simulink model "tg9"  (R2022a)
settings: Solver=ode15s  StartTime=0.0  StopTime=10  MaxStep=0.01  RelTol=1e-3
InitFcn:
  | mecha_param2
  | control_param0
values from neighbouring files (symbols this model uses):
  b0 = 0    [sim_IMMC.m]
  b1 = 1    [sim_IMMC.m]
  back0 = 0    [sim_IMMC.m]
  back1 = 0    [sim_IMMC.m]
  boff = 0    [sim_IMMC.m]
  bon = 0    [sim_IMMC.m]
  c = 0.05    [mecha_param2.m]
  c_jointstop = 0.3 / (pi/180)    (= 17.1887338539)    [mecha_param2.m]
  calctalus = sqrt((L_foot - (DJ1x_foot))^2 + (H_foot-r_cs)^2)    [mecha_param2.m]
  calctoes = sqrt((H_foot-r_cs)^2 + (DJ1x_foot)^2)    [mecha_param2.m]
  corrD = 0.001    [control_param0.m]
  DG_HAT = 0.35    [mecha_param2.m]
  DG_thigh = 0.28    [mecha_param2.m]
  DJ1x_foot = 0.16-r_cs    (= 0.135)    [mecha_param2.m]
  eref = 0.04    [mecha_param2.m]
  FmaxBFSH = 350    [mecha_param2.m]
  FmaxGAS = 1500    [mecha_param2.m]
  FmaxGLU = 1500    [mecha_param2.m]
  FmaxHAM = 3000    [mecha_param2.m]
  FmaxHFL = 2000    [mecha_param2.m]
  FmaxRF = 1200    [mecha_param2.m]
  FmaxSOL = 4000    [mecha_param2.m]
  FmaxTA = 800    [mecha_param2.m]
  FmaxVAS = 6000    [mecha_param2.m]
  g = 9.81    [mecha_param2.m]
  g0 = 0    [sim_IMMC.m]
  g1 = 0    [sim_IMMC.m]
  H_foot = 0.08    [mecha_param2.m]
  In_HAT = 3    [mecha_param2.m]
  In_shank = 0.05    [mecha_param2.m]
  In_thigh = 0.15    [mecha_param2.m]
  K = 5    [mecha_param2.m]
  knee_thigh = [0 0 -(L_thigh/2)]    [mecha_param2.m]
  Kpress = m_HAT * g / DeltaThRef    (= 104967)    [mecha_param2.m]
  L_foot = 0.2    [mecha_param2.m]
  L_HAT = 0.8    [mecha_param2.m]
  L_shank = 0.46    [mecha_param2.m]
  L_thigh = 0.46    [mecha_param2.m]
  LoHAM = table2array(mt('LoHAM', 1))    [control_param0.m]
  LoHFL = table2array(mt('LoHFL', 1))    [control_param0.m]
  longD = longD - corrD    (= 0.019)    [control_param0.m]
  loptBFSH = 0.12    [mecha_param2.m]
  loptGAS = 0.05    [mecha_param2.m]
  loptGLU = 0.11    [mecha_param2.m]
  loptHAM = 0.10    (= 0.1)    [mecha_param2.m]
  loptHFL = 0.11    [mecha_param2.m]
  loptRF = 0.08    [mecha_param2.m]
  loptSOL = 0.04    [mecha_param2.m]
  loptTA = 0.06    [mecha_param2.m]
  loptVAS = 0.08    [mecha_param2.m]
  LoTA = table2array(mt('LoTA', 1))    [control_param0.m]
  lslackBFSH = 0.10    (= 0.1)    [mecha_param2.m]
  lslackGAS = 0.40    (= 0.4)    [mecha_param2.m]
  lslackGLU = 0.13    [mecha_param2.m]
  lslackHAM = 0.31    [mecha_param2.m]
  lslackHFL = 0.10    (= 0.1)    [mecha_param2.m]
  lslackRF = 0.35    [mecha_param2.m]
  lslackSOL = 0.26    [mecha_param2.m]
  lslackTA = 0.24    [mecha_param2.m]
  lslackVAS = 0.23    [mecha_param2.m]
  m_HAT = 53.5    [mecha_param2.m]
  m_shank = 3.5    [mecha_param2.m]
  m_thigh = 8.5    [mecha_param2.m]
  midD = midD - corrD    (= 0.009)    [control_param0.m]
  N = 1.5    [mecha_param2.m]
  nonoff = 0    [control_param0.m]
  phi_a_low = (70) * (pi / 180)    (= 1.2217304764)    [mecha_param2.m]
  phi_a_up = (130) * (pi / 180)    (= 2.26892802759)    [mecha_param2.m]
  phi_dl = 180    [mecha_param2.m]
  phi_h = 230 * (pi / 180)    (= 4.01425727959)    [mecha_param2.m]
  phi_k = 175 * (pi / 180)    (= 3.05432619099)    [mecha_param2.m]
  phictoes = asind((DJ1y_foot-r_cs)/calctoes)    [mecha_param2.m]
  phimaxGASa = 100*pi/180    (= 1.74532925199)    [mecha_param2.m]
  phimaxGASk = 140*pi/180    (= 2.44346095279)    [mecha_param2.m]
  phimaxRFk = 165*pi/180    (= 2.87979326579)    [mecha_param2.m]
  phimaxSOL = 100*pi/180    (= 1.74532925199)    [mecha_param2.m]
  phimaxTA = 80*pi/180    (= 1.3962634016)    [mecha_param2.m]
  phimaxVAS = 165*pi/180    (= 2.87979326579)    [mecha_param2.m]
  phirefBFSH = 160*pi/180    (= 2.79252680319)    [mecha_param2.m]
  phirefGASa = 80*pi/180    (= 1.3962634016)    [mecha_param2.m]
  phirefGASk = 165*pi/180    (= 2.87979326579)    [mecha_param2.m]
  phirefGLU = 120*pi/180    (= 2.09439510239)    [mecha_param2.m]
  phirefHAMh = 150*pi/180    (= 2.61799387799)    [mecha_param2.m]
  phirefHAMk = 180*pi/180    (= 3.14159265359)    [mecha_param2.m]
  phirefHFL = 160*pi/180    (= 2.79252680319)    [mecha_param2.m]
  phirefRFh = 170*pi/180    (= 2.96705972839)    [mecha_param2.m]
  phirefRFk = 125*pi/180    (= 2.18166156499)    [mecha_param2.m]
  phirefSOL = 90*pi/180    (= 1.57079632679)    [mecha_param2.m]
  phirefTA = 110*pi/180    (= 1.91986217719)    [mecha_param2.m]
  phirefVAS = 120*pi/180    (= 2.09439510239)    [mecha_param2.m]
  phiScaleGASa = acos(rGASamin/rGASamax)/(phiminGASa-phimaxGASa)    [mecha_param2.m]
  phiScaleGASk = acos(rGASkmin/rGASkmax)/(phiminGASk-phimaxGASk)    [mecha_param2.m]
  phiScaleRFk = acos(rRFkmin/rRFkmax)/(phiminRFk-phimaxRFk)    [mecha_param2.m]
  phiScaleSOL = acos(rSOLmin/rSOLmax)/(phiminSOL-phimaxSOL)    [mecha_param2.m]
  phiScaleTA = acos(rTAmin/rTAmax)/(phiminTA-phimaxTA)    [mecha_param2.m]
  phiScaleVAS = acos(rVASmin/rVASmax)/(phiminVAS-phimaxVAS)    [mecha_param2.m]
  r1 = 0    [sim_IMMC.m]
  r_cs = 0.025    [mecha_param2.m]
  rBFSH = 0.04    [mecha_param2.m]
  rGASamax = 0.06    [mecha_param2.m]
  rGASkmax = 0.05    [mecha_param2.m]
  rGLU = 0.08    [mecha_param2.m]
  rHAMh = 0.08    [mecha_param2.m]
  rHAMk = 0.05    [mecha_param2.m]
  rHFL = 0.08    [mecha_param2.m]
  rhoBFSH = 0.7    [mecha_param2.m]
  rhoGASa = 0.7    [mecha_param2.m]
  rhoGASk = 0.7    [mecha_param2.m]
  rhoGLU = 0.5    [mecha_param2.m]
  rhoHAMh = 0.5    [mecha_param2.m]
  rhoHAMk = 0.5    [mecha_param2.m]
  rhoHFL = 0.5    [mecha_param2.m]
  rhoRFh = 0.3    [mecha_param2.m]
  rhoRFk = 0.5    [mecha_param2.m]
  rhoSOL = 0.5    [mecha_param2.m]
  rhoTA = 0.7    [mecha_param2.m]
  rhoVAS = 0.6    [mecha_param2.m]
  rRFh = 0.08    [mecha_param2.m]
  rRFkmax = 0.06    [mecha_param2.m]
  rSOLmax = 0.06    [mecha_param2.m]
  ... (+25 more)
undefined symbols (not defined in the file or in its folder): beta11, beta12, beta13, beta14, beta15, beta16, beta21, beta22, beta23, beta24, beta25, beta26, beta31, beta32, beta33, beta34, beta35, beta36, beta41, beta42, beta43, beta44, beta45, beta46, beta51, beta52, beta53, beta54, beta55, beta56, betab1, betab2, betab3, betab4, betab5, betab6, betap11, betap12, betap13, betap14, betap15, betap16, betap21, betap22, betap23, betap24, betap25, betap26, betap31, betap32, betap33, betap34, betap35, betap36, betap41, betap42, betap43, betap44, betap45, betap46 ... (+102)
libraries: sm_lib x89, simulink x72, nesl_utility x58, simulink_extras x18
(part 6 of 12)

== system tg9/Muscle Actuation Layer/L Ankle Joint Limit ==
  note: Right Ankle Soft Limit
  phi [rad] : Inport
  dphi [rad/s] : Inport  Port=2
  Gain : Gain  Gain=c_jointstop
  Gain1 : Gain  Gain=1/w_max_jointstop
  Gain2 : Gain  Gain=-1
  Gain3 : Gain  Gain=c_jointstop
  Interval Test : simulink/Logic and Bit Operations/Interval Test  IntervalClosedRight=on  uplimit=phi_a_up + 40*pi/180  IntervalClosedLeft=on  lowlimit=phi_a_low - 40*pi/180  OutDataTypeStr=boolean
  Logical Operator : Logic  Operator=NOT  AllPortsSameDT=off  OutDataTypeStr=boolean
  Mux : Mux  Inputs=2
  Mux1 : Mux  Inputs=2
  Overextension torque : MATLAB Function  TreatAsAtomicUnit=on
  Overflexion torque : MATLAB Function  TreatAsAtomicUnit=on
  Scope : Scope
  Scope1 : Scope  NumInputPorts=2
  Stop Simulation : Stop
  Sum : Sum  Inputs=|+-
  Sum1 : Sum  Inputs=|+-
  Sum2 : Sum  Inputs=+|+
  overextension angle : Constant  Value=phi_a_up
  overflexion angle : Constant  Value=phi_a_low
  M_stop [Nm] : Outport
  wires:
  phi [rad]/1 -> Sum/1, Interval Test/1, Sum1/1
  overextension angle/1 -> Sum/2
  dphi [rad/s]/1 -> Gain1/1
  Sum/1 -> Gain/1
  Gain1/1 -> Mux1/2, Gain2/1
  Gain/1 -> Mux/1
  Gain2/1 -> Mux/2
  Mux/1 -> Overextension torque/1(u)
  Interval Test/1 -> Logical Operator/1
  Logical Operator/1 -> Scope/1, Stop Simulation/1
  Gain3/1 -> Mux1/1
  Sum1/1 -> Gain3/1
  overflexion angle/1 -> Sum1/2
  Overflexion torque/1(y) -> Sum2/2, Scope1/2
  Mux1/1 -> Overflexion torque/1(u)
  Overextension torque/1(y) -> Scope1/1, Sum2/1
  Sum2/1 -> M_stop [Nm]/1

== system tg9/Muscle Actuation Layer/L BFSH ==
  note: fv
  note: STIM to A
  note: v[vmax] becomes v when *vmax and vce when *lopt
  note: lce is the integration of vce over time using lopt as initial condition
  note: vce
  note: activation
  note: stimulation
  note: Fmax
  note: Fmtc = Fse
  note: outcome fse is a proportion of fmax, because of that, it must be multiplied by fmax in order to get Fse
  note: lceo = lmtu-lslack
  note: lse=lmtu-lce
  note: lse/lslack
  note: lce/lopt
  note: lce
  note: lce
  note: lce
  note: lmtu
  note: lmtu
  note: Left Biceps femoris short-head Musculo-Tendon Unit
  STIM : Inport
  lmtu [m] : Inport  Port=2
  BE force-length relation : Subsystem
  CE force-length relation : Subsystem
  CE inverse force-velocity relation : Subsystem
  Constant : Constant  Value=lslackBFSH
  ECC TransferFcn : simulink_extras/Additional Linear/Transfer Fcn (with initial outputs)  N=[1]  D="[tau  1]"  Y0=preA  U0=0
  Fv = (Fse+Fbe) / (A*Fce+Fpe) : Product  Inputs=*/
  Gain : Gain  Gain=vmaxBFSH*loptBFSH
  Gain1 : Gain  Gain=1/lslackBFSH
  Gain2 : Gain  Gain=1/loptBFSH
  Gain3 : Gain  Gain=FmaxBFSH
  Integrator : Integrator  InitialConditionSource=external  ZeroCross=off
  PE force-length relation : Subsystem
  Product : Product
  SE force-length relation : Subsystem
  Sum : Sum  Inputs=|+-
  Sum1 : Sum  Inputs=|-+
  Sum2 : Sum  Inputs=+|+
  Sum3 : Sum  Inputs=+|+
  excentric branch1 : Fcn  Commented=on  Expr=u(2) * (u(1)>1)*(u(1)<=u(3))
  Fmtc : Outport
  Lce : Outport  Port=2
  Vce : Outport  Port=3
  lse : Outport  Port=4
  A : Outport  Port=5
  fce [Fmax] : Outport  Port=6
  "fse [Fmax}" : Outport  Port=7
  wires:
  CE inverse force-velocity relation/1(v[vmax]) -> Gain/1
  PE force-length relation/1(fpe [Fmax]) -> Sum3/1
  BE force-length relation/1(fbe [Fmax]) -> Sum2/2
  Fv = (Fse+Fbe) / (A*Fce+Fpe)/1 -> CE inverse force-velocity relation/1(Fv[Fmax])
  Sum3/1 -> Fv = (Fse+Fbe) / (A*Fce+Fpe)/2
  Sum2/1 -> Fv = (Fse+Fbe) / (A*Fce+Fpe)/1
  Gain3/1 -> Fmtc/1
  ECC TransferFcn/1 -> Product/2, A/1
  STIM/1 -> ECC TransferFcn/1
  Product/1 -> Sum3/2
  CE force-length relation/1(fce [Fmax]) -> Product/1, fce [Fmax]/1
  SE force-length relation/1(fse [Fmax]) -> Sum2/1, Gain3/1, "fse [Fmax}"/1
  Gain1/1 -> SE force-length relation/1(lse [lslack])
  Gain2/1 -> CE force-length relation/1(lce [lopt]), BE force-length relation/1(lce [lopt]), PE force-length relation/1(lce [lopt])
  Sum/1 -> Gain1/1, lse/1
  Gain/1 -> Integrator/1, Vce/1
  Sum1/1 -> Integrator/2
  Constant/1 -> Sum1/1
  Integrator/1 -> Lce/1, Gain2/1, Sum/2
  lmtu [m]/1 -> Sum/1, Sum1/2

== system tg9/Muscle Actuation Layer/L BFSH Link1 ==
  note: BFSH Attachment
  phi23 [rad] : Inport
  Constant : Constant  Value=lslackBFSH+loptBFSH
  Constant1 : Constant  Value=rBFSH
  Constant2 : Constant  Value=phirefBFSH
  Gain4 : Gain  Gain=rhoBFSH
  Product : Product  RndMeth=Zero
  Sum2 : Sum  Inputs=|+-
  Sum5 : Sum  Inputs=|++
  lmtu [m] : Outport
  lever [m] : Outport  Port=2
  wires:
  Constant/1 -> Sum5/1
  Sum5/1 -> lmtu [m]/1
  Gain4/1 -> Sum5/2
  Product/1 -> Gain4/1
  phi23 [rad]/1 -> Sum2/1
  Constant2/1 -> Sum2/2
  Sum2/1 -> Product/1
  Constant1/1 -> Product/2, lever [m]/1

== system tg9/Muscle Actuation Layer/L BFSH Link2 ==
  note: BFSH Attachment
  phi23 [rad] : Inport
  Constant : Constant  Value=lslackBFSH+loptBFSH
  Constant1 : Constant  Value=rBFSH
  Constant2 : Constant  Value=phirefBFSH
  Gain4 : Gain  Gain=rhoBFSH
  Product : Product  RndMeth=Zero
  Sum2 : Sum  Inputs=|+-
  Sum5 : Sum  Inputs=|++
  lmtu [m] : Outport
  lever [m] : Outport  Port=2
  wires:
  Constant/1 -> Sum5/1
  Sum5/1 -> lmtu [m]/1
  Gain4/1 -> Sum5/2
  Product/1 -> Gain4/1
  phi23 [rad]/1 -> Sum2/1
  Constant2/1 -> Sum2/2
  Sum2/1 -> Product/1
  Constant1/1 -> Product/2, lever [m]/1

== system tg9/Muscle Actuation Layer/L GAS ==
  note: Left Gastrocnemius Musculo-Tendon Unit
  note: lmtu
  note: lmtu
  note: lce
  note: lce
  note: lce
  note: lce/lopt
  note: lse/lslack
  note: lse=lmtu-lce
  note: lceo = lmtu-lslack
  note: outcome fse is a proportion of fmax, because of that, it must be multiplied by fmax in order to get Fse
  note: Fmtc = Fse
  note: Fmax
  note: stimulation
  note: activation
  note: vce
  note: lce is the integration of vce over time using lopt as initial condition
  note: v[vmax] becomes v when *vmax and vce when *lopt
  note: STIM to A
  note: fv
  STIM : Inport
  lmtu [m] : Inport  Port=2
  BE force-length relation : Subsystem
  CE force-length relation : Subsystem
  CE inverse force-velocity relation : Subsystem
  Constant : Constant  Value=lslackGAS
  ECC TransferFcn : simulink_extras/Additional Linear/Transfer Fcn (with initial outputs)  N=[1]  D="[tau  1]"  Y0=preA  U0=0
  Fv = (Fse+Fbe) / (A*Fce+Fpe) : Product  Inputs=*/
  Gain : Gain  Gain=vmaxGAS*loptGAS
  Gain1 : Gain  Gain=1/lslackGAS
  Gain2 : Gain  Gain=1/loptGAS
  Gain3 : Gain  Gain=FmaxGAS
  Integrator : Integrator  InitialConditionSource=external  ZeroCross=off
  PE force-length relation : Subsystem
  Product : Product
  SE force-length relation : Subsystem
  Sum : Sum  Inputs=|+-
  Sum1 : Sum  Inputs=|-+
  Sum2 : Sum  Inputs=+|+
  Sum3 : Sum  Inputs=+|+
  excentric branch1 : Fcn  Commented=on  Expr=u(2) * (u(1)>1)*(u(1)<=u(3))
  Fmtc : Outport
  Lce : Outport  Port=2
  Vce : Outport  Port=3
  lse : Outport  Port=4
  A : Outport  Port=5
  fce [Fmax] : Outport  Port=6
  "fse [Fmax}" : Outport  Port=7
  wires:
  lmtu [m]/1 -> Sum1/2, Sum/1
  Integrator/1 -> Sum/2, Gain2/1, Lce/1
  Constant/1 -> Sum1/1
  Sum1/1 -> Integrator/2
  Gain/1 -> Vce/1, Integrator/1
  Sum/1 -> lse/1, Gain1/1
  Gain2/1 -> PE force-length relation/1(lce [lopt]), BE force-length relation/1(lce [lopt]), CE force-length relation/1(lce [lopt])
  Gain1/1 -> SE force-length relation/1(lse [lslack])
  SE force-length relation/1(fse [Fmax]) -> "fse [Fmax}"/1, Gain3/1, Sum2/1
  CE force-length relation/1(fce [Fmax]) -> Product/1, fce [Fmax]/1
  Product/1 -> Sum3/2
  STIM/1 -> ECC TransferFcn/1
  ECC TransferFcn/1 -> A/1, Product/2
  Gain3/1 -> Fmtc/1
  Sum2/1 -> Fv = (Fse+Fbe) / (A*Fce+Fpe)/1
  Sum3/1 -> Fv = (Fse+Fbe) / (A*Fce+Fpe)/2
  Fv = (Fse+Fbe) / (A*Fce+Fpe)/1 -> CE inverse force-velocity relation/1(Fv[Fmax])
  BE force-length relation/1(fbe [Fmax]) -> Sum2/2
  PE force-length relation/1(fpe [Fmax]) -> Sum3/1
  CE inverse force-velocity relation/1(v[vmax]) -> Gain/1

== system tg9/Muscle Actuation Layer/L GAS Link1 ==
  note: GAS Attachment
  phi23 [rad] : Inport
  phi12 [rad] : Inport  Port=2
  Constant1 : Constant  Value=phimaxGASk
  Constant2 : Constant  Value=phirefGASk
  Constant3 : Constant  Value=phimaxGASa
  Constant4 : Constant  Value=lslackGAS+loptGAS
  Constant5 : Constant  Value=phirefGASa
  Demux : Demux  Outputs=2
  Demux1 : Demux  Outputs=2
  Gain1 : Gain  Gain=rGASkmax
  Gain2 : Gain  Gain=rGASamax
  Gain3 : Gain  Gain=phiScaleGASa
  Gain5 : Gain  Gain=phiScaleGASk
  Gain6 : Gain  Gain=phiScaleGASk
  Gain7 : Gain  Gain=rhoGASk/phiScaleGASk
  Gain8 : Gain  Gain=phiScaleGASa
  Gain9 : Gain  Gain=rhoGASa/phiScaleGASa
  Mux : Mux  Inputs=2
  Mux1 : Mux  Inputs=2
  Sum1 : Sum  Inputs=-+
  Sum2 : Sum  Inputs=|+-
  Sum3 : Sum  Inputs=-+|
  Sum4 : Sum  Inputs=-+
  Sum5 : Sum  Inputs=++-
  Sum6 : Sum  Inputs=|+-
  Sum7 : Sum  Inputs=-+|
  length change term : Trigonometry
  length change term1 : Trigonometry
  offset correction term : Trigonometry
  offset correction term1 : Trigonometry
  variable lever term : Trigonometry  Operator=cos
  variable lever term1 : Trigonometry  Operator=cos
  lmtu [m] : Outport
  lever23 [m] : Outport  Port=2
  lever12 [m] : Outport  Port=3
  wires:
  Sum5/1 -> lmtu [m]/1
  Demux1/2 -> lever12 [m]/1
  Constant4/1 -> Sum5/2
  Demux1/1 -> Gain9/1
  Gain9/1 -> Sum5/3
  Demux/2 -> lever23 [m]/1
  Demux/1 -> Gain7/1
  Gain7/1 -> Sum5/1
  phi23 [rad]/1 -> Sum3/2
  Sum3/1 -> Gain5/1
  Constant1/1 -> Sum3/1, Sum2/2
  Sum2/1 -> Gain6/1
  Constant2/1 -> Sum2/1
  length change term/1 -> Sum1/2
  offset correction term/1 -> Sum1/1
  Sum1/1 -> Mux/1
  variable lever term/1 -> Mux/2
  Mux/1 -> Gain1/1
  Gain1/1 -> Demux/1
  Gain5/1 -> variable lever term/1, length change term/1
  Gain6/1 -> offset correction term/1
  phi12 [rad]/1 -> Sum7/2
  Sum7/1 -> Gain3/1
  Constant3/1 -> Sum7/1, Sum6/2
  Sum6/1 -> Gain8/1
  Constant5/1 -> Sum6/1
  length change term1/1 -> Sum4/2
  offset correction term1/1 -> Sum4/1
  Sum4/1 -> Mux1/1
  variable lever term1/1 -> Mux1/2
  Mux1/1 -> Gain2/1
  Gain2/1 -> Demux1/1
  Gain3/1 -> variable lever term1/1, length change term1/1
  Gain8/1 -> offset correction term1/1

== system tg9/Muscle Actuation Layer/L GAS Link2 ==
  note: GAS Attachment
  phi23 [rad] : Inport
  phi12 [rad] : Inport  Port=2
  Constant1 : Constant  Value=phimaxGASk
  Constant2 : Constant  Value=phirefGASk
  Constant3 : Constant  Value=phimaxGASa
  Constant4 : Constant  Value=lslackGAS+loptGAS
  Constant5 : Constant  Value=phirefGASa
  Demux : Demux  Outputs=2
  Demux1 : Demux  Outputs=2
  Gain1 : Gain  Gain=rGASkmax
  Gain2 : Gain  Gain=rGASamax
  Gain3 : Gain  Gain=phiScaleGASa
  Gain5 : Gain  Gain=phiScaleGASk
  Gain6 : Gain  Gain=phiScaleGASk
  Gain7 : Gain  Gain=rhoGASk/phiScaleGASk
  Gain8 : Gain  Gain=phiScaleGASa
  Gain9 : Gain  Gain=rhoGASa/phiScaleGASa
  Mux : Mux  Inputs=2
  Mux1 : Mux  Inputs=2
  Sum1 : Sum  Inputs=-+
  Sum2 : Sum  Inputs=|+-
  Sum3 : Sum  Inputs=-+|
  Sum4 : Sum  Inputs=-+
  Sum5 : Sum  Inputs=++-
  Sum6 : Sum  Inputs=|+-
  Sum7 : Sum  Inputs=-+|
  length change term : Trigonometry
  length change term1 : Trigonometry
  offset correction term : Trigonometry
  offset correction term1 : Trigonometry
  variable lever term : Trigonometry  Operator=cos
  variable lever term1 : Trigonometry  Operator=cos
  lmtu [m] : Outport
  lever23 [m] : Outport  Port=2
  lever12 [m] : Outport  Port=3
  wires:
  Sum5/1 -> lmtu [m]/1
  Demux1/2 -> lever12 [m]/1
  Constant4/1 -> Sum5/2
  Demux1/1 -> Gain9/1
  Gain9/1 -> Sum5/3
  Demux/2 -> lever23 [m]/1
  Demux/1 -> Gain7/1
  Gain7/1 -> Sum5/1
  phi23 [rad]/1 -> Sum3/2
  Sum3/1 -> Gain5/1
  Constant1/1 -> Sum3/1, Sum2/2
  Sum2/1 -> Gain6/1
  Constant2/1 -> Sum2/1
  length change term/1 -> Sum1/2
  offset correction term/1 -> Sum1/1
  Sum1/1 -> Mux/1
  variable lever term/1 -> Mux/2
  Mux/1 -> Gain1/1
  Gain1/1 -> Demux/1
  Gain5/1 -> variable lever term/1, length change term/1
  Gain6/1 -> offset correction term/1
  phi12 [rad]/1 -> Sum7/2
  Sum7/1 -> Gain3/1
  Constant3/1 -> Sum7/1, Sum6/2
  Sum6/1 -> Gain8/1
  Constant5/1 -> Sum6/1
  length change term1/1 -> Sum4/2
  offset correction term1/1 -> Sum4/1
  Sum4/1 -> Mux1/1
  variable lever term1/1 -> Mux1/2
  Mux1/1 -> Gain2/1
  Gain2/1 -> Demux1/1
  Gain3/1 -> variable lever term1/1, length change term1/1
  Gain8/1 -> offset correction term1/1

== system tg9/Muscle Actuation Layer/L GLU ==
  note: Left Gluteus Musculo-Tendon Unit
  note: lmtu
  note: lmtu
  note: lce
  note: lce
  note: lce
  note: lce/lopt
  note: lse/lslack
  note: lse=lmtu-lce
  note: lceo = lmtu-lslack
  note: outcome fse is a proportion of fmax, because of that, it must be multiplied by fmax in order to get Fse
  note: Fmtc = Fse
  note: Fmax
  note: stimulation
  note: activation
  note: vce
  note: lce is the integration of vce over time using lopt as initial condition
  note: v[vmax] becomes v when *vmax and vce when *lopt
  note: STIM to A
  note: fv
  STIM : Inport
  lmtu [m] : Inport  Port=2
  BE force-length relation : Subsystem
  CE force-length relation : Subsystem
  CE inverse force-velocity relation : Subsystem
  Constant : Constant  Value=lslackGLU
  ECC TransferFcn : simulink_extras/Additional Linear/Transfer Fcn (with initial outputs)  N=[1]  D="[tau  1]"  Y0=preA  U0=0
  Fv = (Fse+Fbe) / (A*Fce+Fpe) : Product  Inputs=*/
  Gain : Gain  Gain=vmaxGLU*loptGLU
  Gain1 : Gain  Gain=1/lslackGLU
  Gain2 : Gain  Gain=1/loptGLU
  Gain3 : Gain  Gain=FmaxGLU
  Integrator : Integrator  InitialConditionSource=external  ZeroCross=off
  PE force-length relation : Subsystem
  Product : Product
  SE force-length relation : Subsystem
  Sum : Sum  Inputs=|+-
  Sum1 : Sum  Inputs=|-+
  Sum2 : Sum  Inputs=+|+
  Sum3 : Sum  Inputs=+|+
  excentric branch1 : Fcn  Commented=on  Expr=u(2) * (u(1)>1)*(u(1)<=u(3))
  Fmtc : Outport
  Lce : Outport  Port=2
  Vce : Outport  Port=3
  lse : Outport  Port=4
  A : Outport  Port=5
  fce [Fmax] : Outport  Port=6
  "fse [Fmax}" : Outport  Port=7
  wires:
  lmtu [m]/1 -> Sum1/2, Sum/1
  Integrator/1 -> Sum/2, Gain2/1, Lce/1
  Constant/1 -> Sum1/1
  Sum1/1 -> Integrator/2
  Gain/1 -> Vce/1, Integrator/1
  Sum/1 -> lse/1, Gain1/1
  Gain2/1 -> PE force-length relation/1(lce [lopt]), BE force-length relation/1(lce [lopt]), CE force-length relation/1(lce [lopt])
  Gain1/1 -> SE force-length relation/1(lse [lslack])
  SE force-length relation/1(fse [Fmax]) -> "fse [Fmax}"/1, Gain3/1, Sum2/1
  CE force-length relation/1(fce [Fmax]) -> Product/1, fce [Fmax]/1
  Product/1 -> Sum3/2
  STIM/1 -> ECC TransferFcn/1
  ECC TransferFcn/1 -> A/1, Product/2
  Gain3/1 -> Fmtc/1
  Sum2/1 -> Fv = (Fse+Fbe) / (A*Fce+Fpe)/1
  Sum3/1 -> Fv = (Fse+Fbe) / (A*Fce+Fpe)/2
  Fv = (Fse+Fbe) / (A*Fce+Fpe)/1 -> CE inverse force-velocity relation/1(Fv[Fmax])
  BE force-length relation/1(fbe [Fmax]) -> Sum2/2
  PE force-length relation/1(fpe [Fmax]) -> Sum3/1
  CE inverse force-velocity relation/1(v[vmax]) -> Gain/1

== system tg9/Muscle Actuation Layer/L GLU Link ==
  note: GLUTEUS Attachment
  phi34 [rad] : Inport
  Constant : Constant  Value=lslackGLU+loptGLU
  Constant1 : Constant  Value=rGLU
  Constant2 : Constant  Value=phirefGLU
  Gain2 : Gain  Gain=rhoGLU
  Product : Product  RndMeth=Zero
  Sum2 : Sum  Inputs=|+-
  Sum5 : Sum  Inputs=|+-
  lmtu [m] : Outport
  lever [m] : Outport  Port=2
  wires:
  Constant/1 -> Sum5/1
  Sum5/1 -> lmtu [m]/1
  Product/1 -> Gain2/1
  phi34 [rad]/1 -> Sum2/1
  Constant2/1 -> Sum2/2
  Sum2/1 -> Product/1
  Constant1/1 -> Product/2, lever [m]/1
  Gain2/1 -> Sum5/2

== system tg9/Muscle Actuation Layer/L GLU Link1 ==
  note: GLUTEUS Attachment
  phi34 [rad] : Inport
  Constant : Constant  Value=lslackGLU+loptGLU
  Constant1 : Constant  Value=rGLU
  Constant2 : Constant  Value=phirefGLU
  Gain2 : Gain  Gain=rhoGLU
  Product : Product  RndMeth=Zero
  Sum2 : Sum  Inputs=|+-
  Sum5 : Sum  Inputs=|+-
  lmtu [m] : Outport
  lever [m] : Outport  Port=2
  wires:
  Constant/1 -> Sum5/1
  Sum5/1 -> lmtu [m]/1
  Product/1 -> Gain2/1
  phi34 [rad]/1 -> Sum2/1
  Constant2/1 -> Sum2/2
  Sum2/1 -> Product/1
  Constant1/1 -> Product/2, lever [m]/1
  Gain2/1 -> Sum5/2

== system tg9/Muscle Actuation Layer/L HAM ==
  note: Left Hamstrings Musculo-Tendon Unit
  note: lmtu
  note: lmtu
  note: lce
  note: lce
  note: lce
  note: lce/lopt
  note: lse/lslack
  note: lse=lmtu-lce
  note: lceo = lmtu-lslack
  note: outcome fse is a proportion of fmax, because of that, it must be multiplied by fmax in order to get Fse
  note: Fmtc = Fse
  note: Fmax
  note: stimulation
  note: activation
  note: vce
  note: lce is the integration of vce over time using lopt as initial condition
  note: v[vmax] becomes v when *vmax and vce when *lopt
  note: STIM to A
  note: fv
  STIM : Inport
  lmtu [m] : Inport  Port=2
  BE force-length relation : Subsystem
  CE force-length relation : Subsystem
  CE inverse force-velocity relation : Subsystem
  Constant : Constant  Value=lslackHAM
  ECC TransferFcn : simulink_extras/Additional Linear/Transfer Fcn (with initial outputs)  N=[1]  D="[tau  1]"  Y0=preA  U0=0
  Fv = (Fse+Fbe) / (A*Fce+Fpe) : Product  Inputs=*/
  Gain : Gain  Gain=vmaxHAM*loptHAM
  Gain1 : Gain  Gain=1/lslackHAM
  Gain2 : Gain  Gain=1/loptHAM
  Gain3 : Gain  Gain=FmaxHAM
  Integrator : Integrator  InitialConditionSource=external  ZeroCross=off
  PE force-length relation : Subsystem
  Product : Product
  SE force-length relation : Subsystem
  Sum : Sum  Inputs=|+-
  Sum1 : Sum  Inputs=|-+
  Sum2 : Sum  Inputs=+|+
  Sum3 : Sum  Inputs=+|+
  excentric branch1 : Fcn  Commented=on  Expr=u(2) * (u(1)>1)*(u(1)<=u(3))
  Fmtc : Outport
  Lce : Outport  Port=2
  Vce : Outport  Port=3
  lse : Outport  Port=4
  A : Outport  Port=5
  fce [Fmax] : Outport  Port=6
  "fse [Fmax}" : Outport  Port=7
  wires:
  lmtu [m]/1 -> Sum1/2, Sum/1
  Integrator/1 -> Sum/2, Gain2/1, Lce/1
  Constant/1 -> Sum1/1
  Sum1/1 -> Integrator/2
  Gain/1 -> Vce/1, Integrator/1
  Sum/1 -> lse/1, Gain1/1
  Gain2/1 -> PE force-length relation/1(lce [lopt]), BE force-length relation/1(lce [lopt]), CE force-length relation/1(lce [lopt])
  Gain1/1 -> SE force-length relation/1(lse [lslack])
  SE force-length relation/1(fse [Fmax]) -> "fse [Fmax}"/1, Gain3/1, Sum2/1
  CE force-length relation/1(fce [Fmax]) -> fce [Fmax]/1, Product/1
  Product/1 -> Sum3/2
  STIM/1 -> ECC TransferFcn/1
  ECC TransferFcn/1 -> A/1, Product/2
  Gain3/1 -> Fmtc/1
  Sum2/1 -> Fv = (Fse+Fbe) / (A*Fce+Fpe)/1
  Sum3/1 -> Fv = (Fse+Fbe) / (A*Fce+Fpe)/2
  Fv = (Fse+Fbe) / (A*Fce+Fpe)/1 -> CE inverse force-velocity relation/1(Fv[Fmax])
  BE force-length relation/1(fbe [Fmax]) -> Sum2/2
  PE force-length relation/1(fpe [Fmax]) -> Sum3/1
  CE inverse force-velocity relation/1(v[vmax]) -> Gain/1

== system tg9/Muscle Actuation Layer/L HAM Link1 ==
  note: HAM Attachment
  phi34 [rad] : Inport
  phi23 [rad] : Inport  Port=2
  Constant1 : Constant  Value=rHAMk
  Constant2 : Constant  Value=phirefHAMk
  Constant3 : Constant  Value=rHAMh
  Constant4 : Constant  Value=lslackHAM+loptHAM
  Constant5 : Constant  Value=phirefHAMh
  Gain2 : Gain  Gain=rhoHAMh
  Gain4 : Gain  Gain=rhoHAMk
  Product : Product  RndMeth=Zero
  Product1 : Product  RndMeth=Zero
  Sum1 : Sum  Inputs=|+-
  Sum4 : Sum  Inputs=|+-
  Sum5 : Sum  Inputs=-++
  lmtu [m] : Outport
  lever34 [m] : Outport  Port=2
  lever23 [m] : Outport  Port=3
  wires:
  Sum5/1 -> lmtu [m]/1
  Constant4/1 -> Sum5/2
  Gain4/1 -> Sum5/3
  Gain2/1 -> Sum5/1
  phi34 [rad]/1 -> Sum4/1
  Constant5/1 -> Sum4/2
  Sum4/1 -> Product/1
  Constant3/1 -> Product/2, lever34 [m]/1
  Product/1 -> Gain2/1
  phi23 [rad]/1 -> Sum1/1
  Constant2/1 -> Sum1/2
  Sum1/1 -> Product1/1
  Constant1/1 -> Product1/2, lever23 [m]/1
  Product1/1 -> Gain4/1

== system tg9/Muscle Actuation Layer/L HAM Link2 ==
  note: HAM Attachment
  phi34 [rad] : Inport
  phi23 [rad] : Inport  Port=2
  Constant1 : Constant  Value=rHAMk
  Constant2 : Constant  Value=phirefHAMk
  Constant3 : Constant  Value=rHAMh
  Constant4 : Constant  Value=lslackHAM+loptHAM
  Constant5 : Constant  Value=phirefHAMh
  Gain2 : Gain  Gain=rhoHAMh
  Gain4 : Gain  Gain=rhoHAMk
  Product : Product  RndMeth=Zero
  Product1 : Product  RndMeth=Zero
  Sum1 : Sum  Inputs=|+-
  Sum4 : Sum  Inputs=|+-
  Sum5 : Sum  Inputs=-++
  lmtu [m] : Outport
  lever34 [m] : Outport  Port=2
  lever23 [m] : Outport  Port=3
  wires:
  Sum5/1 -> lmtu [m]/1
  Constant4/1 -> Sum5/2
  Gain4/1 -> Sum5/3
  Gain2/1 -> Sum5/1
  phi34 [rad]/1 -> Sum4/1
  Constant5/1 -> Sum4/2
  Sum4/1 -> Product/1
  Constant3/1 -> Product/2, lever34 [m]/1
  Product/1 -> Gain2/1
  phi23 [rad]/1 -> Sum1/1
  Constant2/1 -> Sum1/2
  Sum1/1 -> Product1/1
  Constant1/1 -> Product1/2, lever23 [m]/1
  Product1/1 -> Gain4/1

== system tg9/Muscle Actuation Layer/L HFL ==
  note: Left Hip Flexor Group Musculo-Tendon Unit
  note: lmtu
  note: lmtu
  note: lce
  note: lce
  note: lce
  note: lce/lopt
  note: lse/lslack
  note: lse=lmtu-lce
  note: lceo = lmtu-lslack
  note: outcome fse is a proportion of fmax, because of that, it must be multiplied by fmax in order to get Fse
  note: Fmtc = Fse
  note: Fmax
  note: stimulation
  note: activation
  note: vce
  note: lce is the integration of vce over time using lopt as initial condition
  note: v[vmax] becomes v when *vmax and vce when *lopt
  note: STIM to A
  note: fv
  STIM : Inport
  lmtu [m] : Inport  Port=2
  BE force-length relation : Subsystem
  CE force-length relation : Subsystem
  CE inverse force-velocity relation : Subsystem
  Constant : Constant  Value=lslackHFL
  ECC TransferFcn : simulink_extras/Additional Linear/Transfer Fcn (with initial outputs)  N=[1]  D="[tau  1]"  Y0=preA  U0=0
  Fv = (Fse+Fbe) / (A*Fce+Fpe) : Product  Inputs=*/
  Gain : Gain  Gain=vmaxHFL*loptHFL
  Gain1 : Gain  Gain=1/lslackHFL
  Gain2 : Gain  Gain=1/loptHFL
  Gain3 : Gain  Gain=FmaxHFL
  Integrator : Integrator  InitialConditionSource=external  ZeroCross=off
  PE force-length relation : Subsystem
  Product : Product
  SE force-length relation : Subsystem
  Sum : Sum  Inputs=|+-
  Sum1 : Sum  Inputs=|-+
  Sum2 : Sum  Inputs=+|+
  Sum3 : Sum  Inputs=+|+
  excentric branch1 : Fcn  Commented=on  Expr=u(2) * (u(1)>1)*(u(1)<=u(3))
  Fmtc : Outport
  Lce : Outport  Port=2
  Vce : Outport  Port=3
  lse : Outport  Port=4
  A : Outport  Port=5
  fce [Fmax] : Outport  Port=6
  "fse [Fmax}" : Outport  Port=7
  wires:
  lmtu [m]/1 -> Sum1/2, Sum/1
  Integrator/1 -> Sum/2, Gain2/1, Lce/1
  Constant/1 -> Sum1/1
  Sum1/1 -> Integrator/2
  Gain/1 -> Vce/1, Integrator/1
  Sum/1 -> lse/1, Gain1/1
  Gain2/1 -> PE force-length relation/1(lce [lopt]), BE force-length relation/1(lce [lopt]), CE force-length relation/1(lce [lopt])
  Gain1/1 -> SE force-length relation/1(lse [lslack])
  SE force-length relation/1(fse [Fmax]) -> "fse [Fmax}"/1, Gain3/1, Sum2/1
  CE force-length relation/1(fce [Fmax]) -> fce [Fmax]/1, Product/1
  Product/1 -> Sum3/2
  STIM/1 -> ECC TransferFcn/1
  ECC TransferFcn/1 -> A/1, Product/2
  Gain3/1 -> Fmtc/1
  Sum2/1 -> Fv = (Fse+Fbe) / (A*Fce+Fpe)/1
  Sum3/1 -> Fv = (Fse+Fbe) / (A*Fce+Fpe)/2
  Fv = (Fse+Fbe) / (A*Fce+Fpe)/1 -> CE inverse force-velocity relation/1(Fv[Fmax])
  BE force-length relation/1(fbe [Fmax]) -> Sum2/2
  PE force-length relation/1(fpe [Fmax]) -> Sum3/1
  CE inverse force-velocity relation/1(v[vmax]) -> Gain/1

== system tg9/Muscle Actuation Layer/L HFL Link1 ==
  note: HFL Attachment
  phi34 [rad] : Inport
  Constant : Constant  Value=lslackHFL+loptHFL
  Constant1 : Constant  Value=rHFL
  Constant2 : Constant  Value=phirefHFL
  Gain2 : Gain  Gain=rhoHFL
  Product : Product  RndMeth=Zero
  Sum2 : Sum  Inputs=|+-
  Sum5 : Sum  Inputs=|++
  lmtu [m] : Outport
  lever [m] : Outport  Port=2
  wires:
  Constant/1 -> Sum5/1
  Sum5/1 -> lmtu [m]/1
  Product/1 -> Gain2/1
  phi34 [rad]/1 -> Sum2/1
  Constant2/1 -> Sum2/2
  Sum2/1 -> Product/1
  Constant1/1 -> Product/2, lever [m]/1
  Gain2/1 -> Sum5/2

== system tg9/Muscle Actuation Layer/L HFL Link2 ==
  note: HFL Attachment
  phi34 [rad] : Inport
  Constant : Constant  Value=lslackHFL+loptHFL
  Constant1 : Constant  Value=rHFL
  Constant2 : Constant  Value=phirefHFL
  Gain2 : Gain  Gain=rhoHFL
  Product : Product  RndMeth=Zero
  Sum2 : Sum  Inputs=|+-
  Sum5 : Sum  Inputs=|++
  lmtu [m] : Outport
  lever [m] : Outport  Port=2
  wires:
  Constant/1 -> Sum5/1
  Sum5/1 -> lmtu [m]/1
  Product/1 -> Gain2/1
  phi34 [rad]/1 -> Sum2/1
  Constant2/1 -> Sum2/2
  Sum2/1 -> Product/1
  Constant1/1 -> Product/2, lever [m]/1
  Gain2/1 -> Sum5/2

== system tg9/Muscle Actuation Layer/L Hip Joint Limits ==
  note: Left Hip Soft Limit
  phi hip [rad] : Inport
  dphi hip [rad/s] : Inport  Port=2
  Gain : Gain  Gain=c_jointstop
  Gain1 : Gain  Gain=1/w_max_jointstop
  Gain2 : Gain  Gain=-1
  Interval Test : simulink/Logic and Bit Operations/Interval Test  IntervalClosedRight=on  uplimit=phi_h + 30*pi/180  IntervalClosedLeft=on  lowlimit=10*pi/180  OutDataTypeStr=boolean
  Logical Operator : Logic  Operator=NOT  AllPortsSameDT=off  OutDataTypeStr=boolean
  Mux : Mux  Inputs=2
  Overextension torque : MATLAB Function  TreatAsAtomicUnit=on
  Scope : Scope  NumInputPorts=2
  Stop Simulation : Stop
  Sum : Sum  Inputs=|+-
  overextension angle : Constant  Value=phi_h
  M_stop [Nm] : Outport
  wires:
  phi hip [rad]/1 -> Interval Test/1, Sum/1
  overextension angle/1 -> Sum/2
  dphi hip [rad/s]/1 -> Gain1/1
  Sum/1 -> Gain/1
  Gain1/1 -> Gain2/1
  Gain/1 -> Mux/1
  Gain2/1 -> Mux/2
  Mux/1 -> Overextension torque/1(u)
  Interval Test/1 -> Logical Operator/1
  Logical Operator/1 -> Scope/2, Stop Simulation/1
  Overextension torque/1(y) -> Scope/1, M_stop [Nm]/1

== system tg9/Muscle Actuation Layer/L Knee Joint Limits ==
  note: Left Knee Soft Limit
  phi [rad] : Inport
  dphi [rad/s] : Inport  Port=2
  Gain : Gain  Gain=c_jointstop
  Gain1 : Gain  Gain=1/w_max_jointstop
  Gain2 : Gain  Gain=-1
  Interval Test : simulink/Logic and Bit Operations/Interval Test  IntervalClosedRight=on  uplimit=185*pi/180  IntervalClosedLeft=on  lowlimit=40*pi/180  OutDataTypeStr=boolean
  Logical Operator : Logic  Operator=NOT  AllPortsSameDT=off  OutDataTypeStr=boolean
  Mux : Mux  Inputs=2
  Overextension torque : MATLAB Function  TreatAsAtomicUnit=on
  Stop Simulation : Stop
  Sum : Sum  Inputs=|+-
  overextension angle : Constant  Value=phi_k
  M_stop [Nm] : Outport
  tag scope: Knee_pain=global
  wires:
  phi [rad]/1 -> Interval Test/1, Sum/1
  overextension angle/1 -> Sum/2
  dphi [rad/s]/1 -> Gain1/1
  Sum/1 -> Gain/1
  Gain1/1 -> Gain2/1
  Gain/1 -> Mux/1
  Gain2/1 -> Mux/2
  Mux/1 -> Overextension torque/1(u)
  Overextension torque/1(y) -> [Knee_pain], M_stop [Nm]/1
  Interval Test/1 -> Logical Operator/1
  Logical Operator/1 -> Stop Simulation/1

== system tg9/Muscle Actuation Layer/L RF ==
  note: fv
  note: STIM to A
  note: v[vmax] becomes v when *vmax and vce when *lopt
  note: lce is the integration of vce over time using lopt as initial condition
  note: vce
  note: activation
  note: stimulation
  note: Fmax
  note: Fmtc = Fse
  note: outcome fse is a proportion of fmax, because of that, it must be multiplied by fmax in order to get Fse
  note: lceo = lmtu-lslack
  note: lse=lmtu-lce
  note: lse/lslack
  note: lce/lopt
  note: lce
  note: lce
  note: lce
  note: lmtu
  note: lmtu
  note: Left Vastus Musculo-Tendon Unit
  STIM : Inport
  lmtu [m] : Inport  Port=2
  BE force-length relation : Subsystem
  CE force-length relation : Subsystem
  CE inverse force-velocity relation : Subsystem
  Constant : Constant  Value=lslackRF
  ECC TransferFcn : simulink_extras/Additional Linear/Transfer Fcn (with initial outputs)  N=[1]  D="[tau  1]"  Y0=preA  U0=0
  Fv = (Fse+Fbe) / (A*Fce+Fpe) : Product  Inputs=*/
  Gain : Gain  Gain=vmaxRF*loptRF
  Gain1 : Gain  Gain=1/lslackRF
  Gain2 : Gain  Gain=1/loptRF
  Gain3 : Gain  Gain=FmaxRF
  Integrator : Integrator  InitialConditionSource=external  ZeroCross=off
  PE force-length relation : Subsystem
  Product : Product
  SE force-length relation : Subsystem
  Sum : Sum  Inputs=|+-
  Sum1 : Sum  Inputs=|-+
  Sum2 : Sum  Inputs=+|+
  Sum3 : Sum  Inputs=+|+
  excentric branch1 : Fcn  Commented=on  Expr=u(2) * (u(1)>1)*(u(1)<=u(3))
  Fmtc : Outport
  Lce : Outport  Port=2
  Vce : Outport  Port=3
  lse : Outport  Port=4
  A : Outport  Port=5
  fce [Fmax] : Outport  Port=6
  "fse [Fmax}" : Outport  Port=7
  wires:
  CE inverse force-velocity relation/1(v[vmax]) -> Gain/1
  PE force-length relation/1(fpe [Fmax]) -> Sum3/1
  BE force-length relation/1(fbe [Fmax]) -> Sum2/2
  Fv = (Fse+Fbe) / (A*Fce+Fpe)/1 -> CE inverse force-velocity relation/1(Fv[Fmax])
  Sum3/1 -> Fv = (Fse+Fbe) / (A*Fce+Fpe)/2
  Sum2/1 -> Fv = (Fse+Fbe) / (A*Fce+Fpe)/1
  Gain3/1 -> Fmtc/1
  ECC TransferFcn/1 -> Product/2, A/1
  STIM/1 -> ECC TransferFcn/1
  Product/1 -> Sum3/2
  CE force-length relation/1(fce [Fmax]) -> Product/1, fce [Fmax]/1
  SE force-length relation/1(fse [Fmax]) -> Sum2/1, Gain3/1, "fse [Fmax}"/1
  Gain1/1 -> SE force-length relation/1(lse [lslack])
  Gain2/1 -> CE force-length relation/1(lce [lopt]), BE force-length relation/1(lce [lopt]), PE force-length relation/1(lce [lopt])
  Sum/1 -> Gain1/1, lse/1
  Gain/1 -> Integrator/1, Vce/1
  Sum1/1 -> Integrator/2
  Constant/1 -> Sum1/1
  Integrator/1 -> Lce/1, Gain2/1, Sum/2
  lmtu [m]/1 -> Sum/1, Sum1/2

== system tg9/Muscle Actuation Layer/L RF Link1 ==
  note: RF Attachment
  phi34 [rad] : Inport
  phi23 [rad] : Inport  Port=2
  Constant1 : Constant  Value=phimaxRFk
  Constant2 : Constant  Value=phirefRFk
  Constant3 : Constant  Value=rRFh
  Constant4 : Constant  Value=lslackRF+loptRF
  Constant5 : Constant  Value=phirefRFh
  Demux : Demux  Outputs=2
  Gain1 : Gain  Gain=rRFkmax
  Gain2 : Gain  Gain=rhoRFh
  Gain3 : Gain  Gain=phiScaleRFk
  Gain4 : Gain  Gain=rhoRFk/phiScaleRFk
  Gain5 : Gain  Gain=phiScaleRFk
  Mux : Mux  Inputs=2
  Product : Product  RndMeth=Zero
  Sum1 : Sum  Inputs=-+
  Sum2 : Sum  Inputs=|+-
  Sum3 : Sum  Inputs=-+|
  Sum4 : Sum  Inputs=|+-
  Sum5 : Sum  Inputs=++-
  length change term : Trigonometry
  offset correction term : Trigonometry
  variable lever term : Trigonometry  Operator=cos
  lmtu [m] : Outport
  lever34 [m] : Outport  Port=2
  lever23 [m] : Outport  Port=3
  wires:
  Sum5/1 -> lmtu [m]/1
  Constant4/1 -> Sum5/2
  Gain4/1 -> Sum5/3
  Gain2/1 -> Sum5/1
  phi34 [rad]/1 -> Sum4/1
  Constant5/1 -> Sum4/2
  Sum4/1 -> Product/1
  Constant3/1 -> Product/2, lever34 [m]/1
  Product/1 -> Gain2/1
  phi23 [rad]/1 -> Sum3/2
  Sum3/1 -> Gain3/1
  Constant1/1 -> Sum3/1, Sum2/2
  Sum2/1 -> Gain5/1
  Constant2/1 -> Sum2/1
  length change term/1 -> Sum1/2
  offset correction term/1 -> Sum1/1
  Sum1/1 -> Mux/1
  variable lever term/1 -> Mux/2
  Mux/1 -> Gain1/1
  Gain1/1 -> Demux/1
  Demux/2 -> lever23 [m]/1
  Demux/1 -> Gain4/1
  Gain3/1 -> variable lever term/1, length change term/1
  Gain5/1 -> offset correction term/1

== system tg9/Muscle Actuation Layer/L RF Link2 ==
  note: RF Attachment
  phi34 [rad] : Inport
  phi23 [rad] : Inport  Port=2
  Constant1 : Constant  Value=phimaxRFk
  Constant2 : Constant  Value=phirefRFk
  Constant3 : Constant  Value=rRFh
  Constant4 : Constant  Value=lslackRF+loptRF
  Constant5 : Constant  Value=phirefRFh
  Demux : Demux  Outputs=2
  Gain1 : Gain  Gain=rRFkmax
  Gain2 : Gain  Gain=rhoRFh
  Gain3 : Gain  Gain=phiScaleRFk
  Gain4 : Gain  Gain=rhoRFk/phiScaleRFk
  Gain5 : Gain  Gain=phiScaleRFk
  Mux : Mux  Inputs=2
  Product : Product  RndMeth=Zero
  Sum1 : Sum  Inputs=-+
  Sum2 : Sum  Inputs=|+-
  Sum3 : Sum  Inputs=-+|
  Sum4 : Sum  Inputs=|+-
  Sum5 : Sum  Inputs=++-
  length change term : Trigonometry
  offset correction term : Trigonometry
  variable lever term : Trigonometry  Operator=cos
  lmtu [m] : Outport
  lever34 [m] : Outport  Port=2
  lever23 [m] : Outport  Port=3
  wires:
  Sum5/1 -> lmtu [m]/1
  Constant4/1 -> Sum5/2
  Gain4/1 -> Sum5/3
  Gain2/1 -> Sum5/1
  phi34 [rad]/1 -> Sum4/1
  Constant5/1 -> Sum4/2
  Sum4/1 -> Product/1
  Constant3/1 -> Product/2, lever34 [m]/1
  Product/1 -> Gain2/1
  phi23 [rad]/1 -> Sum3/2
  Sum3/1 -> Gain3/1
  Constant1/1 -> Sum3/1, Sum2/2
  Sum2/1 -> Gain5/1
  Constant2/1 -> Sum2/1
  length change term/1 -> Sum1/2
  offset correction term/1 -> Sum1/1
  Sum1/1 -> Mux/1
  variable lever term/1 -> Mux/2
  Mux/1 -> Gain1/1
  Gain1/1 -> Demux/1
  Demux/2 -> lever23 [m]/1
  Demux/1 -> Gain4/1
  Gain3/1 -> variable lever term/1, length change term/1
  Gain5/1 -> offset correction term/1

== system tg9/Muscle Actuation Layer/L SOL ==
  note: Left Soleus Musculo-Tendon Unit
  note: lmtu
  note: lmtu
  note: lce
  note: lce
  note: lce
  note: lce/lopt
  note: lse/lslack
  note: lse=lmtu-lce
  note: lceo = lmtu-lslack
  note: outcome fse is a proportion of fmax, because of that, it must be multiplied by fmax in order to get Fse
  note: Fmtc = Fse
  note: Fmax
  note: stimulation
  note: activation
  note: vce
  note: lce is the integration of vce over time using lopt as initial condition
  note: v[vmax] becomes v when *vmax and vce when *lopt
  note: STIM to A
  note: fv
  STIM : Inport
  lmtu [m] : Inport  Port=2
  BE force-length relation : Subsystem
  CE force-length relation : Subsystem
  CE inverse force-velocity relation : Subsystem
  Constant : Constant  Value=lslackSOL
  ECC TransferFcn : simulink_extras/Additional Linear/Transfer Fcn (with initial outputs)  N=[1]  D="[tau  1]"  Y0=preA  U0=0
  Fv = (Fse+Fbe) / (A*Fce+Fpe) : Product  Inputs=*/
  Gain : Gain  Gain=vmaxSOL*loptSOL
  Gain1 : Gain  Gain=1/lslackSOL
  Gain2 : Gain  Gain=1/loptSOL
  Gain3 : Gain  Gain=FmaxSOL
  Integrator : Integrator  InitialConditionSource=external  ZeroCross=off
  PE force-length relation : Subsystem
  Product : Product
  SE force-length relation : Subsystem
  Sum : Sum  Inputs=|+-
  Sum1 : Sum  Inputs=|-+
  Sum2 : Sum  Inputs=+|+
  Sum3 : Sum  Inputs=+|+
  excentric branch1 : Fcn  Commented=on  Expr=u(2) * (u(1)>1)*(u(1)<=u(3))
  Fmtc : Outport
  Lce : Outport  Port=2
  Vce : Outport  Port=3
  lse : Outport  Port=4
  A : Outport  Port=5
  fce [Fmax] : Outport  Port=6
  "fse [Fmax}" : Outport  Port=7
  wires:
  lmtu [m]/1 -> Sum1/2, Sum/1
  Integrator/1 -> Sum/2, Gain2/1, Lce/1
  Constant/1 -> Sum1/1
  Sum1/1 -> Integrator/2
  Gain/1 -> Vce/1, Integrator/1
  Sum/1 -> lse/1, Gain1/1
  Gain2/1 -> PE force-length relation/1(lce [lopt]), BE force-length relation/1(lce [lopt]), CE force-length relation/1(lce [lopt])
  Gain1/1 -> SE force-length relation/1(lse [lslack])
  SE force-length relation/1(fse [Fmax]) -> "fse [Fmax}"/1, Gain3/1, Sum2/1
  CE force-length relation/1(fce [Fmax]) -> fce [Fmax]/1, Product/1
  Product/1 -> Sum3/2
  STIM/1 -> ECC TransferFcn/1
  ECC TransferFcn/1 -> A/1, Product/2
  Gain3/1 -> Fmtc/1
  Sum2/1 -> Fv = (Fse+Fbe) / (A*Fce+Fpe)/1
  Sum3/1 -> Fv = (Fse+Fbe) / (A*Fce+Fpe)/2
  Fv = (Fse+Fbe) / (A*Fce+Fpe)/1 -> CE inverse force-velocity relation/1(Fv[Fmax])
  BE force-length relation/1(fbe [Fmax]) -> Sum2/2
  PE force-length relation/1(fpe [Fmax]) -> Sum3/1
  CE inverse force-velocity relation/1(v[vmax]) -> Gain/1

== system tg9/Muscle Actuation Layer/L SOL Link1 ==
  note: Soleus Attachment
  phi12 [rad] : Inport
  Constant : Constant  Value=lslackSOL+loptSOL
  Constant3 : Constant  Value=phimaxSOL
  Constant5 : Constant  Value=phirefSOL
  Demux1 : Demux  Outputs=2
  Gain2 : Gain  Gain=rSOLmax
  Gain3 : Gain  Gain=phiScaleSOL
  Gain8 : Gain  Gain=phiScaleSOL
  Gain9 : Gain  Gain=rhoSOL/phiScaleSOL
  Mux1 : Mux  Inputs=2
  Sum4 : Sum  Inputs=-+
  Sum5 : Sum  Inputs=|+-
  Sum6 : Sum  Inputs=|+-
  Sum7 : Sum  Inputs=-+|
  length change term1 : Trigonometry
  offset correction term1 : Trigonometry
  variable lever term1 : Trigonometry  Operator=cos
  lmtc [m] : Outport
  lever [m] : Outport  Port=2
  wires:
  Constant/1 -> Sum5/1
  Sum5/1 -> lmtc [m]/1
  Gain9/1 -> Sum5/2
  Demux1/1 -> Gain9/1
  Demux1/2 -> lever [m]/1
  phi12 [rad]/1 -> Sum7/2
  Sum7/1 -> Gain3/1
  Constant3/1 -> Sum7/1, Sum6/2
  Sum6/1 -> Gain8/1
  Constant5/1 -> Sum6/1
  length change term1/1 -> Sum4/2
  offset correction term1/1 -> Sum4/1
  Sum4/1 -> Mux1/1
  variable lever term1/1 -> Mux1/2
  Mux1/1 -> Gain2/1
  Gain2/1 -> Demux1/1
  Gain3/1 -> variable lever term1/1, length change term1/1
  Gain8/1 -> offset correction term1/1

== system tg9/Muscle Actuation Layer/L SOL Link2 ==
  note: Soleus Attachment
  phi12 [rad] : Inport
  Constant : Constant  Value=lslackSOL+loptSOL
  Constant3 : Constant  Value=phimaxSOL
  Constant5 : Constant  Value=phirefSOL
  Demux1 : Demux  Outputs=2
  Gain2 : Gain  Gain=rSOLmax
  Gain3 : Gain  Gain=phiScaleSOL
  Gain8 : Gain  Gain=phiScaleSOL
  Gain9 : Gain  Gain=rhoSOL/phiScaleSOL
  Mux1 : Mux  Inputs=2
  Sum4 : Sum  Inputs=-+
  Sum5 : Sum  Inputs=|+-
  Sum6 : Sum  Inputs=|+-
  Sum7 : Sum  Inputs=-+|
  length change term1 : Trigonometry
  offset correction term1 : Trigonometry
  variable lever term1 : Trigonometry  Operator=cos
  lmtc [m] : Outport
  lever [m] : Outport  Port=2
  wires:
  Constant/1 -> Sum5/1
  Sum5/1 -> lmtc [m]/1
  Gain9/1 -> Sum5/2
  Demux1/1 -> Gain9/1
  Demux1/2 -> lever [m]/1
  phi12 [rad]/1 -> Sum7/2
  Sum7/1 -> Gain3/1
  Constant3/1 -> Sum7/1, Sum6/2
  Sum6/1 -> Gain8/1
  Constant5/1 -> Sum6/1
  length change term1/1 -> Sum4/2
  offset correction term1/1 -> Sum4/1
  Sum4/1 -> Mux1/1
  variable lever term1/1 -> Mux1/2
  Mux1/1 -> Gain2/1
  Gain2/1 -> Demux1/1
  Gain3/1 -> variable lever term1/1, length change term1/1
  Gain8/1 -> offset correction term1/1

== system tg9/Muscle Actuation Layer/L TA ==
  note: Left Tibialis Anterior Musculo-Tendon Unit
  note: lmtu
  note: lmtu
  note: lce
  note: lce
  note: lce
  note: lce/lopt
  note: lse/lslack
  note: lse=lmtu-lce
  note: lceo = lmtu-lslack
  note: outcome fse is a proportion of fmax, because of that, it must be multiplied by fmax in order to get Fse
  note: Fmtc = Fse
  note: Fmax
  note: stimulation
  note: activation
  note: vce
  note: lce is the integration of vce over time using lopt as initial condition
  note: v[vmax] becomes v when *vmax and vce when *lopt
  note: STIM to A
  note: fv
  STIM : Inport
  lmtu [m] : Inport  Port=2
  BE force-length relation : Subsystem
  CE force-length relation : Subsystem
  CE inverse force-velocity relation : Subsystem
  Constant : Constant  Value=lslackTA
  ECC TransferFcn : simulink_extras/Additional Linear/Transfer Fcn (with initial outputs)  N=[1]  D="[tau  1]"  Y0=preA  U0=0
  Fv = (Fse+Fbe) / (A*Fce+Fpe) : Product  Inputs=*/
  Gain : Gain  Gain=vmaxTA*loptTA
  Gain1 : Gain  Gain=1/lslackTA
  Gain2 : Gain  Gain=1/loptTA
  Gain3 : Gain  Gain=FmaxTA
  Integrator : Integrator  InitialConditionSource=external  ZeroCross=off
  PE force-length relation : Subsystem
  Product : Product
  SE force-length relation : Subsystem
  Sum : Sum  Inputs=|+-
  Sum1 : Sum  Inputs=|-+
  Sum2 : Sum  Inputs=+|+
  Sum3 : Sum  Inputs=+|+
  excentric branch1 : Fcn  Commented=on  Expr=u(2) * (u(1)>1)*(u(1)<=u(3))
  Fmtc : Outport
  Lce : Outport  Port=2
  Vce : Outport  Port=3
  lse : Outport  Port=4
  A : Outport  Port=5
  fce [Fmax] : Outport  Port=6
  "fse [Fmax}" : Outport  Port=7
  wires:
  lmtu [m]/1 -> Sum1/2, Sum/1
  Integrator/1 -> Sum/2, Gain2/1, Lce/1
  Constant/1 -> Sum1/1
  Sum1/1 -> Integrator/2
  Gain/1 -> Vce/1, Integrator/1
  Sum/1 -> lse/1, Gain1/1
  Gain2/1 -> PE force-length relation/1(lce [lopt]), BE force-length relation/1(lce [lopt]), CE force-length relation/1(lce [lopt])
  Gain1/1 -> SE force-length relation/1(lse [lslack])
  SE force-length relation/1(fse [Fmax]) -> "fse [Fmax}"/1, Gain3/1, Sum2/1
  CE force-length relation/1(fce [Fmax]) -> fce [Fmax]/1, Product/1
  Product/1 -> Sum3/2
  STIM/1 -> ECC TransferFcn/1
  ECC TransferFcn/1 -> A/1, Product/2
  Gain3/1 -> Fmtc/1
  Sum2/1 -> Fv = (Fse+Fbe) / (A*Fce+Fpe)/1
  Sum3/1 -> Fv = (Fse+Fbe) / (A*Fce+Fpe)/2
  Fv = (Fse+Fbe) / (A*Fce+Fpe)/1 -> CE inverse force-velocity relation/1(Fv[Fmax])
  BE force-length relation/1(fbe [Fmax]) -> Sum2/2
  PE force-length relation/1(fpe [Fmax]) -> Sum3/1
  CE inverse force-velocity relation/1(v[vmax]) -> Gain/1

== system tg9/Muscle Actuation Layer/L TA Link1 ==
  note: Muscle Length and Moment Arm
  phi12 [rad] : Inport
  Constant : Constant  Value=lslackTA+loptTA
  Constant3 : Constant  Value=phimaxTA
  Constant5 : Constant  Value=phirefTA
  Demux1 : Demux  Outputs=2
  Gain2 : Gain  Gain=rTAmax
  Gain3 : Gain  Gain=phiScaleTA
  Gain8 : Gain  Gain=phiScaleTA
  Gain9 : Gain  Gain=rhoTA/phiScaleTA
  Mux1 : Mux  Inputs=2
  Sum4 : Sum  Inputs=-+
  Sum5 : Sum  Inputs=|++
  Sum6 : Sum  Inputs=|+-
  Sum7 : Sum  Inputs=-+|
  length change term1 : Trigonometry
  offset correction term1 : Trigonometry
  variable lever term1 : Trigonometry  Operator=cos
  lmtc [m] : Outport
  lever [m] : Outport  Port=2
  wires:
  Constant/1 -> Sum5/1
  Sum5/1 -> lmtc [m]/1
  Gain9/1 -> Sum5/2
  Demux1/1 -> Gain9/1
  Demux1/2 -> lever [m]/1
  phi12 [rad]/1 -> Sum7/2
  Sum7/1 -> Gain3/1
  Constant3/1 -> Sum7/1, Sum6/2
  Sum6/1 -> Gain8/1
  Constant5/1 -> Sum6/1
  length change term1/1 -> Sum4/2
  offset correction term1/1 -> Sum4/1
  Sum4/1 -> Mux1/1
  variable lever term1/1 -> Mux1/2
  Mux1/1 -> Gain2/1
  Gain2/1 -> Demux1/1
  Gain3/1 -> variable lever term1/1, length change term1/1
  Gain8/1 -> offset correction term1/1

== system tg9/Muscle Actuation Layer/L TA Link2 ==
  note: Muscle Length and Moment Arm
  phi12 [rad] : Inport
  Constant : Constant  Value=lslackTA+loptTA
  Constant3 : Constant  Value=phimaxTA
  Constant5 : Constant  Value=phirefTA
  Demux1 : Demux  Outputs=2
  Gain2 : Gain  Gain=rTAmax
  Gain3 : Gain  Gain=phiScaleTA
  Gain8 : Gain  Gain=phiScaleTA
  Gain9 : Gain  Gain=rhoTA/phiScaleTA
  Mux1 : Mux  Inputs=2
  Sum4 : Sum  Inputs=-+
  Sum5 : Sum  Inputs=|++
  Sum6 : Sum  Inputs=|+-
  Sum7 : Sum  Inputs=-+|
  length change term1 : Trigonometry
  offset correction term1 : Trigonometry
  variable lever term1 : Trigonometry  Operator=cos
  lmtc [m] : Outport
  lever [m] : Outport  Port=2
  wires:
  Constant/1 -> Sum5/1
  Sum5/1 -> lmtc [m]/1
  Gain9/1 -> Sum5/2
  Demux1/1 -> Gain9/1
  Demux1/2 -> lever [m]/1
  phi12 [rad]/1 -> Sum7/2
  Sum7/1 -> Gain3/1
  Constant3/1 -> Sum7/1, Sum6/2
  Sum6/1 -> Gain8/1
  Constant5/1 -> Sum6/1
  length change term1/1 -> Sum4/2
  offset correction term1/1 -> Sum4/1
  Sum4/1 -> Mux1/1
  variable lever term1/1 -> Mux1/2
  Mux1/1 -> Gain2/1
  Gain2/1 -> Demux1/1
  Gain3/1 -> variable lever term1/1, length change term1/1
  Gain8/1 -> offset correction term1/1
